simulink model "AvonGasTurbineController"  (R2024b)
settings: Solver=ode45  StartTime=0.0  StopTime=3000  FixedStep=1  RelTol=1e-3  EnableMultiTasking=on
InitFcn:
  | warning off
libraries: slpidlib x3, simulink x2
(part 2 of 2)

== system AvonGasTurbineController/Subsystem/Subsystem4/cooling 1 ==
  cooling_air_temp : Inport
  cooling_air_flow : Inport  Port=2
  hot_gas_flow : Inport  Port=3
  hot_gas_temp : Inport  Port=4
  "     1" : Product  RndMeth=Zero
  "     2" : Product  Inputs=3  RndMeth=Zero
  "     4" : Product  Inputs=3  RndMeth=Zero
  . : Product  Inputs=*/  RndMeth=Zero
  Cp Temp : Subsystem
  Cp Temp air : Subsystem
  Cp Temp hot gas : Subsystem
  Integrator : Integrator  InitialCondition=765+273.15+12  LimitOutput=on  UpperSaturationLimit=1250+273.15  LowerSaturationLimit=600+273.15
  Memory : Memory  InitialCondition=750+273.15
  Scope1 : Scope
  Sum1 : Sum  Inputs=2
  Sum2 : Sum  Inputs=2
  Sum6 : Sum  Inputs=|+-
  time constant : Gain  Gain=1/3.6
  temp gas : Outport
  gas_flow : Outport  Port=2
  wires:
  hot_gas_temp/1 -> Cp Temp hot gas/1(Tinlet), "     4"/2
  hot_gas_flow/1 -> Sum1/1, "     4"/1
  Cp Temp hot gas/1(Cp(T)) -> "     4"/3
  cooling_air_temp/1 -> Cp Temp air/1(Tinlet), "     2"/2
  cooling_air_flow/1 -> Sum1/2, "     2"/1
  Cp Temp air/1(Cp(T)) -> "     2"/3
  "     2"/1 -> Sum2/1
  "     4"/1 -> Sum2/2
  Sum2/1 -> ./1
  Cp Temp/1(Cp(T)) -> "     1"/2
  Memory/1 -> Cp Temp/1(Tinlet)
  "     1"/1 -> ./2
  ./1 -> Sum6/1
  time constant/1 -> Integrator/1
  Sum6/1 -> time constant/1
  Integrator/1 -> temp gas/1, Scope1/1, Sum6/2, Memory/1
  Sum1/1 -> "     1"/1, gas_flow/1

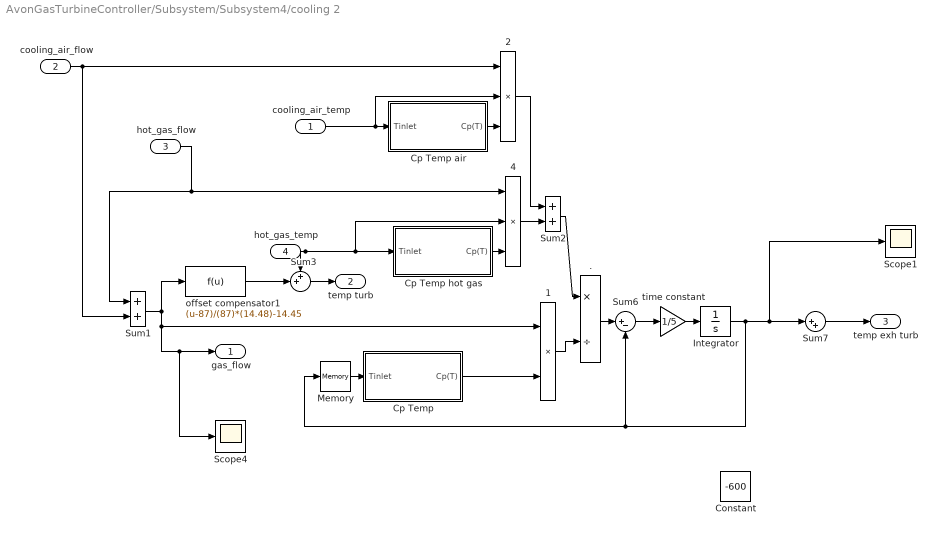
== system AvonGasTurbineController/Subsystem/Subsystem4/cooling 2 ==
  cooling_air_temp : Inport
  cooling_air_flow : Inport  Port=2
  hot_gas_flow : Inport  Port=3
  hot_gas_temp : Inport  Port=4
  "     1" : Product  RndMeth=Zero
  "     2" : Product  Inputs=3  RndMeth=Zero
  "     4" : Product  Inputs=3  RndMeth=Zero
  . : Product  Inputs=*/  RndMeth=Zero
  Constant : Constant  Value=-600
  Cp Temp : Subsystem
  Cp Temp air : Subsystem
  Cp Temp hot gas : Subsystem
  Integrator : Integrator  InitialCondition=1204.4  LimitOutput=on  UpperSaturationLimit=2000  LowerSaturationLimit=100
  Memory : Memory  InitialCondition=500+273.15
  Scope1 : Scope
  Scope4 : Scope
  Sum1 : Sum  Inputs=2
  Sum2 : Sum  Inputs=2
  Sum3 : Sum  Inputs=++|
  Sum6 : Sum  Inputs=|+-
  Sum7 : Sum  Inputs=|++
  offset compensator1 : Fcn  Expr=(u-87)/(87)*(14.48)-14.45
  time constant : Gain  Gain=1/5
  gas_flow : Outport
  temp turb : Outport  Port=2
  temp exh turb : Outport  Port=3
  wires:
  Sum6/1 -> time constant/1
  time constant/1 -> Integrator/1
  ./1 -> Sum6/1
  "     1"/1 -> ./2
  Memory/1 -> Cp Temp/1(Tinlet)
  Cp Temp/1(Cp(T)) -> "     1"/2
  Sum1/1 -> Scope4/1, gas_flow/1, "     1"/1, offset compensator1/1
  Sum2/1 -> ./1
  "     4"/1 -> Sum2/2
  "     2"/1 -> Sum2/1
  Cp Temp air/1(Cp(T)) -> "     2"/3
  cooling_air_flow/1 -> "     2"/1, Sum1/2
  cooling_air_temp/1 -> "     2"/2, Cp Temp air/1(Tinlet)
  Cp Temp hot gas/1(Cp(T)) -> "     4"/3
  hot_gas_flow/1 -> "     4"/1, Sum1/1
  hot_gas_temp/1 -> "     4"/2, Cp Temp hot gas/1(Tinlet), Sum3/1
  Integrator/1 -> Sum7/1, Scope1/1, Sum6/2, Memory/1
  Sum3/1 -> temp turb/1
  offset compensator1/1 -> Sum3/2
  Sum7/1 -> temp exh turb/1

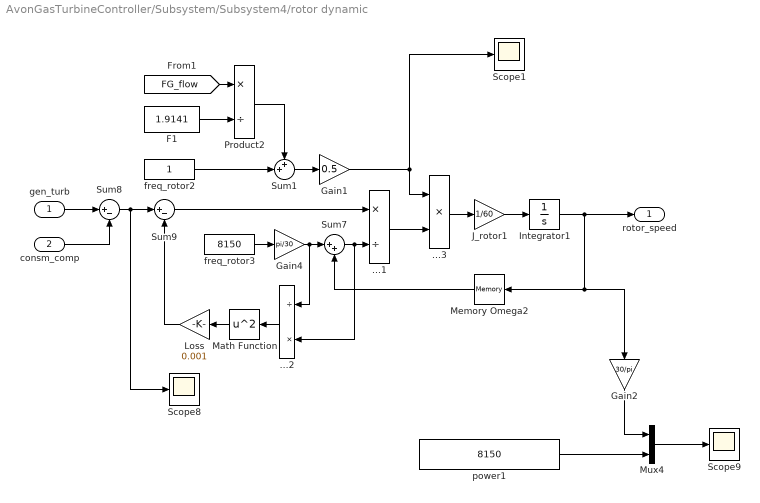
== system AvonGasTurbineController/Subsystem/Subsystem4/rotor dynamic  ==
  gen_turb : Inport
  consm_comp : Inport  Port=2
  ...1 : Product  Inputs=*/
  ...2 : Product  Inputs=/*
  ...3 : Product
  F1 : Constant  Value=1.9141
  Gain1 : Gain  Gain=0.5
  Gain2 : Gain  Gain=30/pi
  Gain4 : Gain  Gain=pi/30
  Integrator1 : Integrator  InitialCondition=pi/30*7250  LimitOutput=on  UpperSaturationLimit=1200  LowerSaturationLimit=0.01
  J_rotor1 : Gain  Gain=1/60
  Loss : Gain  Gain=0.001
  Math Function : Math  Operator=square  SignedPower=on
  Memory Omega2 : Memory  InitialCondition=pi/30*7250
  Mux4 : Mux  Inputs=2
  Product2 : Product  Inputs=*/
  Scope1 : Scope
  Scope8 : Scope
  Scope9 : Scope
  Sum1 : Sum  Inputs=++|
  Sum7 : Sum  Inputs=|++
  Sum8 : Sum  Inputs=|+-
  Sum9 : Sum  Inputs=|+-
  freq_rotor2 : Constant
  freq_rotor3 : Constant  Value=8150
  power1 : Constant  Value=8150
  rotor_speed : Outport
  wires:
  F1/1 -> Product2/2
  Memory Omega2/1 -> Sum7/2
  Gain4/1 -> ...2/1, Sum7/1
  Sum7/1 -> ...2/2, ...1/2
  [FG_flow] -> Product2/1
  freq_rotor3/1 -> Gain4/1
  J_rotor1/1 -> Integrator1/1
  Loss/1 -> Sum9/2
  consm_comp/1 -> Sum8/2
  Sum8/1 -> Scope8/1, Sum9/1
  ...2/1 -> Math Function/1
  Math Function/1 -> Loss/1
  Integrator1/1 -> Gain2/1, Memory Omega2/1, rotor_speed/1
  power1/1 -> Mux4/2
  Mux4/1 -> Scope9/1
  Gain2/1 -> Mux4/1
  gen_turb/1 -> Sum8/1
  Sum9/1 -> ...1/1
  ...1/1 -> ...3/2
  ...3/1 -> J_rotor1/1
  Product2/1 -> Sum1/1
  Gain1/1 -> Scope1/1, ...3/1
  freq_rotor2/1 -> Sum1/2
  Sum1/1 -> Gain1/1

== system AvonGasTurbineController/Subsystem/comp_temp1/Cp @Cop Outlet ==
  Tinlet : Inport
  Cp : Fcn  Expr=(3.355+5.75*1e-4*u(1)-1600*u(1)^(-2))*0.28714  SampleTime=1
  oC-----> K : Fcn  Expr=(u(1)+273.15)  SampleTime=1
  Cp(T) : Outport
  wires:
  oC-----> K/1 -> Cp/1
  Cp/1 -> Cp(T)/1
  Tinlet/1 -> oC-----> K/1

== system AvonGasTurbineController/Subsystem/comp_temp1/Cp_com_in ==
  humidity ratio : Inport
  pressuer : Inport  Port=2
  temp. : Inport  Port=3
  .1 : Product  RndMeth=Zero
  .2 : Product  RndMeth=Zero
  Cp dry air : Subsystem
  Cp steam : Subsystem
  R dry air : Constant  Value=0.287
  R steam : Constant  Value=0.4615
  Specific humidity : Subsystem
  Sum1 : Sum  Inputs=++|
  Sum4 : Sum  Inputs=|++
  Cp : Outport
  Rwet : Outport  Port=2
  wires:
  .1/1 -> Sum4/1
  Specific humidity/1(y) -> .2/2, .1/1
  Cp steam/1(Cp(T)) -> .1/2
  Cp dry air/1(Cp(T)) -> Sum4/2
  humidity ratio/1 -> Specific humidity/1(humidity)
  pressuer/1 -> Specific humidity/2(Press_kPa)
  Sum4/1 -> Cp/1
  temp./1 -> Specific humidity/3(temp), Cp steam/1(Tinlet), Cp dry air/1(Tinlet)
  R steam/1 -> .2/1
  .2/1 -> Sum1/2
  Sum1/1 -> Rwet/1
  R dry air/1 -> Sum1/1

== system AvonGasTurbineController/Subsystem/Combustor1/combustion chamber 1/ Cp dry air  ==
  Tinlet : Inport
  Cp : Fcn  Expr=(3.355+5.75*1e-4*u(1)-1600*u(1)^(-2))*0.28714  SampleTime=1
  Cp(T) : Outport
  wires:
  Tinlet/1 -> Cp/1
  Cp/1 -> Cp(T)/1

== system AvonGasTurbineController/Subsystem/Combustor1/combustion chamber 1/Cp Hot Gas  ==
  Tinlet : Inport
  Cp : Fcn  Expr=(3.355+5.75*1e-4*u(1)-1600*u(1)^(-2))*0.28714  SampleTime=1
  Cp(T) : Outport
  wires:
  Tinlet/1 -> Cp/1  "Kelvin"
  Cp/1 -> Cp(T)/1

== system AvonGasTurbineController/Subsystem/Combustor1/combustion chamber 1/Cp fuel ==
  Tinlet : Inport
  Cp : Fcn  Expr=(1.702+9.081*1e-3*u(1)-2.164*1e-6*u(1)^2)*0.5183  SampleTime=1
  oC-----> K : Fcn  Expr=(u(1)+273.15)  SampleTime=1
  Cp(T) : Outport
  wires:
  oC-----> K/1 -> Cp/1
  Cp/1 -> Cp(T)/1
  Tinlet/1 -> oC-----> K/1

== system AvonGasTurbineController/Subsystem/FG MCV model1/CV model chamber 2/Cp FG ==
  Tinlet : Inport
  Cp : Fcn  Expr=(1.702+9.081*1e-3*u(1)-2.164*1e-6*u(1)^2)*0.5183  SampleTime=1
  oC-----> K : Fcn  Expr=(u(1)+273.15)  SampleTime=1
  Cp(T) : Outport
  wires:
  oC-----> K/1 -> Cp/1
  Cp/1 -> Cp(T)/1
  Tinlet/1 -> oC-----> K/1

== system AvonGasTurbineController/Subsystem/FG MCV model1/CV model chamber 2/density FG ==
  FG_prss : Inport
  FG_temp : Inport  Port=2
  1+0.257*Pr-0.533*Pr/Tr : Fcn  Expr=1+0.257*u(1)-0.533*u(1)/u(2)
  Constant3 : Constant  Value=273.15
  Mux : Mux  Inputs=2
  Sum2 : Sum  Inputs=|++
  Tcr : Constant  Value=191
  Tnormal : Constant  Value=273.15+15
  Tnormal/T : Product  Inputs=*/  RndMeth=Zero
  Zn : Constant  Value=0.9974
  density @ n.c.1 : Gain  Gain=0.78862
  density @ n.c.2 : Gain  Gain=1/14.89
  p/pcr : Product  Inputs=*/  RndMeth=Zero
  p/pnormal1 : Product  Inputs=/*  RndMeth=Zero
  p1 : Product  Inputs=3  RndMeth=Zero
  pcr : Constant  Value=4640
  pnormal2 : Constant  Value=101.3
  t/Tc : Product  Inputs=*/  RndMeth=Zero
  z correction : Product  Inputs=/*  RndMeth=Zero
  density : Outport
  wires:
  Tnormal/1 -> Tnormal/T/1
  Constant3/1 -> Sum2/2
  Sum2/1 -> Tnormal/T/2, t/Tc/1
  pcr/1 -> p/pcr/2
  Tcr/1 -> t/Tc/2
  Zn/1 -> z correction/2
  FG_temp/1 -> Sum2/1
  p/pcr/1 -> Mux/1  "pr"
  t/Tc/1 -> Mux/2  "Tr"
  density @ n.c.2/1 -> density/1
  z correction/1 -> p1/3
  Mux/1 -> 1+0.257*Pr-0.533*Pr/Tr/1
  1+0.257*Pr-0.533*Pr/Tr/1 -> z correction/1
  FG_prss/1 -> p/pnormal1/2, p/pcr/1
  pnormal2/1 -> p/pnormal1/1
  p/pnormal1/1 -> p1/2
  p1/1 -> density @ n.c.1/1
  density @ n.c.1/1 -> density @ n.c.2/1
  Tnormal/T/1 -> p1/1

== system AvonGasTurbineController/Subsystem/FG MCV model1/Subsystem1/Z ==
  T : Inport
  P : Inport  Port=2
  1+0.257*Pr-0.533*Pr/Tr1 : Fcn  Expr=1+0.257*u(1)-0.533*u(1)/u(2)
  Mux5 : Mux  Inputs=2
  Tcr1 : Constant  Value=191
  p/pcr1 : Product  Inputs=*/  RndMeth=Zero
  pcr1 : Constant  Value=4640
  t/Tc1 : Product  Inputs=*/  RndMeth=Zero
  Z : Outport
  wires:
  Mux5/1 -> 1+0.257*Pr-0.533*Pr/Tr1/1
  P/1 -> p/pcr1/1
  T/1 -> t/Tc1/1
  Tcr1/1 -> t/Tc1/2
  1+0.257*Pr-0.533*Pr/Tr1/1 -> Z/1
  t/Tc1/1 -> Mux5/2  "Tr"
  pcr1/1 -> p/pcr1/2
  p/pcr1/1 -> Mux5/1  "pr"

== system AvonGasTurbineController/Subsystem/Subsystem3/Turbine section/hot_air ==
  Tinlet : Inport
  Cp(T) : Fcn  Expr=(3.355+5.75*1e-4*u(1)-1600*u(1)^(-2))*0.28714  SampleTime=1
  Cp(P1,T1) : Outport
  wires:
  Tinlet/1 -> Cp(T)/1
  Cp(T)/1 -> Cp(P1,T1)/1

== system AvonGasTurbineController/Subsystem/Subsystem4/Turbine section/hot_air ==
  Tinlet : Inport
  Cp(T) : Fcn  Expr=(3.355+5.75*1e-4*u(1)-1600*u(1)^(-2))*0.28714  SampleTime=1
  Cp(P1,T1) : Outport
  wires:
  Cp(T)/1 -> Cp(P1,T1)/1
  Tinlet/1 -> Cp(T)/1

== system AvonGasTurbineController/Subsystem/Subsystem4/cooling 1/Cp Temp ==
  Tinlet : Inport
  Cp : Fcn  Expr=(3.355+5.75*1e-4*u(1)-1600*u(1)^(-2))*0.28714  SampleTime=1
  Cp(T) : Outport
  wires:
  Cp/1 -> Cp(T)/1
  Tinlet/1 -> Cp/1  "Kelvin"

== system AvonGasTurbineController/Subsystem/Subsystem4/cooling 1/Cp Temp air ==
  Tinlet : Inport
  Cp : Fcn  Expr=(3.355+5.75*1e-4*u(1)-1600*u(1)^(-2))*0.28714  SampleTime=1
  Cp(T) : Outport
  wires:
  Tinlet/1 -> Cp/1  "Kelvin"
  Cp/1 -> Cp(T)/1

== system AvonGasTurbineController/Subsystem/Subsystem4/cooling 1/Cp Temp hot gas ==
  Tinlet : Inport
  Cp : Fcn  Expr=(3.355+5.75*1e-4*u(1)-1600*u(1)^(-2))*0.28714  SampleTime=1
  Cp(T) : Outport
  wires:
  Cp/1 -> Cp(T)/1
  Tinlet/1 -> Cp/1  "Kelvin"

== system AvonGasTurbineController/Subsystem/Subsystem4/cooling 2/Cp Temp ==
  Tinlet : Inport
  Cp : Fcn  Expr=(3.355+5.75*1e-4*u(1)-1600*u(1)^(-2))*0.28714  SampleTime=1
  Cp(T) : Outport
  wires:
  Tinlet/1 -> Cp/1  "Kelvin"
  Cp/1 -> Cp(T)/1

== system AvonGasTurbineController/Subsystem/Subsystem4/cooling 2/Cp Temp air ==
  Tinlet : Inport
  Cp : Fcn  Expr=(3.355+5.75*1e-4*u(1)-1600*u(1)^(-2))*0.28714  SampleTime=1
  Cp(T) : Outport
  wires:
  Cp/1 -> Cp(T)/1
  Tinlet/1 -> Cp/1  "Kelvin"

== system AvonGasTurbineController/Subsystem/Subsystem4/cooling 2/Cp Temp hot gas ==
  Tinlet : Inport
  Cp : Fcn  Expr=(3.355+5.75*1e-4*u(1)-1600*u(1)^(-2))*0.28714  SampleTime=1
  Cp(T) : Outport
  wires:
  Tinlet/1 -> Cp/1  "Kelvin"
  Cp/1 -> Cp(T)/1

== system AvonGasTurbineController/Subsystem/comp_temp1/Cp_com_in/Cp dry air ==
  Tinlet : Inport
  Cp : Fcn  Expr=(3.355+5.75*1e-4*u(1)-1600*u(1)^(-2))*0.28714  SampleTime=1
  Cp(T) : Outport
  wires:
  Cp/1 -> Cp(T)/1
  Tinlet/1 -> Cp/1

== system AvonGasTurbineController/Subsystem/comp_temp1/Cp_com_in/Cp steam ==
  Tinlet : Inport
  Cp : Fcn  Expr=(3.47+1.45*1e-3*u(1)+1.21*1e4*u(1)^(-2))*0.4615  SampleTime=1
  Cp(T) : Outport
  wires:
  Tinlet/1 -> Cp/1
  Cp/1 -> Cp(T)/1

== system AvonGasTurbineController/Subsystem/comp_temp1/Cp_com_in/Specific humidity ==
  humidity : Inport
  Press_kPa : Inport  Port=2
  temp : Inport  Port=3
  1/100 : Gain  Gain=0.01
  Ps (saturation pressure) : Fcn  Expr=((u-200.5754)/81.4934)^6.1556  SampleTime=1
  Scope11 : Scope
  "Specific humidity " : Gain  Gain=0.6219
  Sum : Sum  Inputs=-+
  x : Product  RndMeth=Zero
  x1 : Product  Inputs=*/  RndMeth=Zero
  y : Outport
  wires:
  Ps (saturation pressure)/1 -> Scope11/1, x/1
  "Specific humidity "/1 -> y/1
  x1/1 -> "Specific humidity "/1
  Sum/1 -> x1/2
  Press_kPa/1 -> Sum/2
  x/1 -> x1/1, Sum/1  "pv"
  1/100/1 -> x/2
  humidity/1 -> 1/100/1
  temp/1 -> Ps (saturation pressure)/1
